simulink model "My_gfm_battery_sil_2_2"  (R2018b)
settings: Solver=ode45  StartTime=0.0  StopTime=30  MaxStep=1e-4  RelTol=1e-3
PreLoadFcn:
  | modelDir = fileparts(get_param(bdroot,'FileName'));
  | 
  | load_system(fullfile(modelDir,'controls_element_lib.slx'));
  | load_system(fullfile(modelDir,'test_sequence_lib.slx'));
InitFcn:
  | close all;
  | clear all;
  | clc;
  | 
  | % frequency nominals
  | F_NOM = 60;
  | W_NOM = 2 * pi * F_NOM;
  | 
  | % base values relative to inverter
  | % --------------------------------
  | VLL_INV_NOM = 480;
  | P_INV_NOM = 1e6;
  | Q_INV_NOM = 0.5e6;
  | S_INV_NOM = sqrt(P_INV_NOM^2 + Q_INV_NOM^2);
  | 
  | I_INV_BASE = S_INV_NOM/(sqrt(3)*VLL_INV_NOM);
  | Z_INV_BASE = VLL_INV_NOM^2/S_INV_NOM;
  | L_INV_BASE = Z_INV_BASE / W_NOM;
  | C_INV_BASE = 1 / (Z_INV_BASE * W_NOM);
  | 
  | % nominal ratings for Plant model
  | % --------------------------------------
  | INVERTER_COUNT = 100;
  | 
  | VLV_NOM = VLL_INV_NOM;
  | VMV_NOM = 35e3;
  | VHV_NOM = 230e3;
  | S_PLANT = INVERTER_COUNT * S_INV_NOM;
  | 
  | N_GSU = VHV_NOM/VMV_NOM;
  | N_MVT = VMV_NOM/VLV_NOM;
  | 
  | I_LV_BASE = S_PLANT/(sqrt(3)*VLV_NOM);
  | I_MV_BASE = S_PLANT/(sqrt(3)*VMV_NOM);
  | I_HV_BASE = S_PLANT/(sqrt(3)*VHV_NOM);
  | 
  | Z_LV_BASE = VLV_NOM^2/S_PLANT;
  | Z_MV_BASE = VMV_NOM^2/S_PLANT;
  | Z_HV_BASE = VHV_NOM^2/S_PLANT;
  | 
  | L_LV_BASE = Z_LV_BASE / W_NOM;
  | L_MV_BASE = Z_MV_BASE / W_NOM;
  | L_HV_BASE = Z_HV_BASE / W_NOM;
  | C_LV_BASE = 1 / (Z_LV_BASE * W_NOM);
  | C_MV_BASE = 1 / (Z_MV_BASE * W_NOM);
  | C_HV_BASE = 1 / (Z_HV_BASE * W_NOM);
  | 
  | % nominal ratings for Grid model
  | % --------------------------------------
  | VGRID_NOM = VHV_NOM;
  | S_GRID = 2*S_PLANT;
  | I_HV_BASE = S_GRID/(sqrt(3)*VGRID_NOM);
  | Z_GRID_BASE = VGRID_NOM^2/S_GRID;
  | L_GRID_BASE = Z_GRID_BASE / W_NOM;
  | C_GRID_BASE = 1 / (Z_GRID_BASE * W_NOM);
undefined symbols (not defined in the file): j
libraries: simulink x74, controls_element_lib x20, test_sequence_lib x12
(part 9 of 9)

== system My_gfm_battery_sil_2_2/My Inverter Controller 1/My_machineModel_A1/rotor model ==
  p_mechanical : Inport
  p_electrical : Inport  Port=2
  Constant : Constant  Value=nominalFrequency
  HPF (wDamperDecoupler) : TransferFcn  Commented=on  Numerator=[0.3 0]  Denominator=[0.3 1]
  HPF (wDamperDecoupler) 1 : Subsystem
  Integrator1 : Integrator  LimitOutput=on  UpperSaturationLimit=5  LowerSaturationLimit=-5
  Sum : Sum  Inputs=++|
  Sum2 : Sum  Inputs=|+-
  Sum3 : Sum  Inputs=|+-
  k_damp : Gain  Gain=kDamper*SRated
  k_inertia : Gain  Gain=(nominalFrequency/2)/(inertialConstant*SRated)
  oscillator_3ph : Subsystem
  osc[3] : Outport  VectorParamsAs1DForOutWhenUnconnected=on
  f_rotor : Outport  Port=2  VectorParamsAs1DForOutWhenUnconnected=on
  wires:
  Constant/1 -> Sum/1
  Sum/1 -> oscillator_3ph/1(f), f_rotor/1
  k_damp/1 -> Sum2/2
  Integrator1/1 -> HPF (wDamperDecoupler) 1/1(in), Sum/2
  p_mechanical/1 -> Sum3/1
  Sum3/1 -> Sum2/1
  p_electrical/1 -> Sum3/2
  HPF (wDamperDecoupler) 1/1(out) -> k_damp/1
  oscillator_3ph/1(osc[3]) -> osc[3]/1
  k_inertia/1 -> Integrator1/1
  Sum2/1 -> k_inertia/1

== system My_gfm_battery_sil_2_2/My Inverter Controller 1/My_machineModel_A1/voltage analyzer ==
  osc[3] : Inport
  v_terminal : Inport  Port=2
  Complex to Magnitude-Angle : ComplexToMagnitudeAngle
  Complex to Real-Imag : ComplexToRealImag
  Conj : Math  Operator=conj  SaturateOnIntegerOverflow=on
  Product1 : Product
  Product2 : Product
  Real-Imag to Complex1 : RealImagToComplex
  Sum of Elements1 : Sum  Inputs=+
  Sum of Elements2 : Sum  Inputs=+
  Terminator : Terminator
  Transfer Fcn : TransferFcn  Denominator=[0.02 1]
  Transfer Fcn1 : TransferFcn  Denominator=[0.02 1]
  over_sqrt(3) : Gain  Gain=1/sqrt(3)
  over_sqrt(3)1 : Gain  Gain=1/sqrt(3)
  sqrt(2) : Gain  Gain=sqrt(2)
  Vd : Outport  VectorParamsAs1DForOutWhenUnconnected=on
  Vq : Outport  Port=2  VectorParamsAs1DForOutWhenUnconnected=on
  Vt_Mag : Outport  Port=3  VectorParamsAs1DForOutWhenUnconnected=on
  wires:
  Transfer Fcn/1 -> Real-Imag to Complex1/2, Vq/1  "Vq"
  osc[3]/1 -> Conj/1
  Transfer Fcn1/1 -> Real-Imag to Complex1/1, Vd/1  "Vd"
  over_sqrt(3)1/1 -> Transfer Fcn1/1
  over_sqrt(3)/1 -> Transfer Fcn/1
  Complex to Real-Imag/1 -> Product2/1
  Complex to Real-Imag/2 -> Product1/1
  Sum of Elements2/1 -> over_sqrt(3)1/1
  v_terminal/1 -> Product2/2, Product1/2
  Product1/1 -> Sum of Elements1/1
  Sum of Elements1/1 -> over_sqrt(3)/1
  sqrt(2)/1 -> Complex to Real-Imag/1
  Conj/1 -> sqrt(2)/1
  Product2/1 -> Sum of Elements2/1
  Complex to Magnitude-Angle/1 -> Vt_Mag/1  "Vt"
  Real-Imag to Complex1/1 -> Complex to Magnitude-Angle/1  "Vd"
  Complex to Magnitude-Angle/2 -> Terminator/1

== system My_gfm_battery_sil_2_2/ac Network with MVT (native math)/OLTC/LPF3 ==
  1 : Inport
  1/10 : Gain  Gain=1/10
  Integrator : Integrator  InitialCondition=1
  Sum4 : Sum  Inputs=|+-
  Out1 : Outport  VectorParamsAs1DForOutWhenUnconnected=on
  wires:
  1/10/1 -> Integrator/1
  Integrator/1 -> Sum4/2, Out1/1
  1/1 -> Sum4/1
  Sum4/1 -> 1/10/1

== system My_gfm_battery_sil_2_2/ac Network with MVT (native math)/OLTC1/LPF3 ==
  1 : Inport
  1/10 : Gain  Gain=1/10
  Integrator : Integrator  InitialCondition=1
  Sum4 : Sum  Inputs=|+-
  Out1 : Outport  VectorParamsAs1DForOutWhenUnconnected=on
  wires:
  1/10/1 -> Integrator/1
  Integrator/1 -> Sum4/2, Out1/1
  1/1 -> Sum4/1
  Sum4/1 -> 1/10/1

== system My_gfm_battery_sil_2_2/My Inverter Controller /My_acMonitor_A/Analyzer_V/complex_LPF ==
  note: This was needed because Simulink complains when using transfer functions directly on arrays or complex numbers.
  In1 : Inport
  Complex to Real-Imag : ComplexToRealImag
  Gain2 : Gain  Gain=1/tau
  Gain3 : Gain  Gain=1/tau
  Integrator : Integrator
  Integrator1 : Integrator
  Real-Imag to Complex : RealImagToComplex
  Sum : Sum  Inputs=|+-
  Sum1 : Sum  Inputs=|+-
  Out1 : Outport  VectorParamsAs1DForOutWhenUnconnected=on
  wires:
  Real-Imag to Complex/1 -> Out1/1
  In1/1 -> Complex to Real-Imag/1
  Complex to Real-Imag/1 -> Sum/1
  Integrator/1 -> Real-Imag to Complex/1, Sum/2
  Sum1/1 -> Gain3/1
  Complex to Real-Imag/2 -> Sum1/1
  Gain2/1 -> Integrator/1
  Sum/1 -> Gain2/1
  Integrator1/1 -> Sum1/2, Real-Imag to Complex/2
  Gain3/1 -> Integrator1/1

== system My_gfm_battery_sil_2_2/My Inverter Controller /My_acMonitor_A/Analyzer_V1/complex_LPF ==
  note: This was needed because Simulink complains when using transfer functions directly on arrays or complex numbers.
  In1 : Inport
  Complex to Real-Imag : ComplexToRealImag
  Gain2 : Gain  Gain=1/tau
  Gain3 : Gain  Gain=1/tau
  Integrator : Integrator
  Integrator1 : Integrator
  Real-Imag to Complex : RealImagToComplex
  Sum : Sum  Inputs=|+-
  Sum1 : Sum  Inputs=|+-
  Out1 : Outport  VectorParamsAs1DForOutWhenUnconnected=on
  wires:
  Real-Imag to Complex/1 -> Out1/1
  In1/1 -> Complex to Real-Imag/1
  Complex to Real-Imag/1 -> Sum/1
  Integrator/1 -> Real-Imag to Complex/1, Sum/2
  Sum1/1 -> Gain3/1
  Complex to Real-Imag/2 -> Sum1/1
  Gain2/1 -> Integrator/1
  Sum/1 -> Gain2/1
  Integrator1/1 -> Sum1/2, Real-Imag to Complex/2
  Gain3/1 -> Integrator1/1

== system My_gfm_battery_sil_2_2/My Inverter Controller /My_acMonitor_A/PLL_3ph/oscillator_3ph ==
  f : Inport
  Cos : Trigonometry  Operator=cos
  Gain : Gain  Gain=2*pi
  Integrator : Integrator
  Real-Imag to Complex : RealImagToComplex
  Sin : Trigonometry
  Sum1 : Sum  Inputs=|++
  phase_shift : Constant  Value=[0 -1/3 -2/3]
  osc[3] : Outport  VectorParamsAs1DForOutWhenUnconnected=on
  wires:
  Sum1/1 -> Gain/1
  phase_shift/1 -> Sum1/2
  Sin/1 -> Real-Imag to Complex/2
  Integrator/1 -> Sum1/1
  Gain/1 -> Sin/1, Cos/1
  Cos/1 -> Real-Imag to Complex/1
  Real-Imag to Complex/1 -> osc[3]/1
  f/1 -> Integrator/1

== system My_gfm_battery_sil_2_2/My Inverter Controller /My_currentLimiting_B/Current_foldback1/LPF  ==
  In : Inport
  1/0.01 : Gain  Gain=1/0.01
  Integrator : Integrator
  Sum3 : Sum  Inputs=|+-
  Out : Outport  VectorParamsAs1DForOutWhenUnconnected=on
  wires:
  Integrator/1 -> Out/1, Sum3/2
  Sum3/1 -> 1/0.01/1
  In/1 -> Sum3/1
  1/0.01/1 -> Integrator/1

== system My_gfm_battery_sil_2_2/My Inverter Controller /My_machineModel_A/AVR/ Saturation ==
  In : Inport
  Complex to Real-Imag : ComplexToRealImag
  Real-Imag to Complex3 : RealImagToComplex
  Saturation3 : Saturate  UpperLimit=0.1*VllRated  LowerLimit=-0.1*VllRated
  Saturation4 : Saturate  UpperLimit=0.1*VllRated  LowerLimit=-0.1*VllRated
  Out : Outport
  wires:
  Complex to Real-Imag/1 -> Saturation3/1
  Saturation4/1 -> Real-Imag to Complex3/2
  Complex to Real-Imag/2 -> Saturation4/1
  Saturation3/1 -> Real-Imag to Complex3/1
  In/1 -> Complex to Real-Imag/1
  Real-Imag to Complex3/1 -> Out/1

== system My_gfm_battery_sil_2_2/My Inverter Controller /My_machineModel_A/AVR/LPF ==
  In : Inport
  1/tauMeas : Gain  Gain=1/tauMeas
  Integrator : Integrator
  Sum3 : Sum  Inputs=|+-
  Out : Outport  VectorParamsAs1DForOutWhenUnconnected=on
  wires:
  Integrator/1 -> Out/1, Sum3/2
  Sum3/1 -> 1/tauMeas/1
  In/1 -> Sum3/1
  1/tauMeas/1 -> Integrator/1

== system My_gfm_battery_sil_2_2/My Inverter Controller /My_machineModel_A/AVR/LPF  ==
  In : Inport
  1/tauMeas : Gain  Gain=1/tauMeas
  Integrator : Integrator
  Sum3 : Sum  Inputs=|+-
  Out : Outport  VectorParamsAs1DForOutWhenUnconnected=on
  wires:
  Integrator/1 -> Out/1, Sum3/2
  Sum3/1 -> 1/tauMeas/1
  In/1 -> Sum3/1
  1/tauMeas/1 -> Integrator/1

== system My_gfm_battery_sil_2_2/My Inverter Controller /My_machineModel_A/AVR/LPF   ==
  In : Inport
  1/tauMeas : Gain  Gain=1/tauMeas
  Integrator : Integrator
  Sum3 : Sum  Inputs=|+-
  Out : Outport  VectorParamsAs1DForOutWhenUnconnected=on
  wires:
  Integrator/1 -> Out/1, Sum3/2
  Sum3/1 -> 1/tauMeas/1
  In/1 -> Sum3/1
  1/tauMeas/1 -> Integrator/1

== system My_gfm_battery_sil_2_2/My Inverter Controller /My_machineModel_A/AVR/assymmetric filter ==
  note: The saturation block is configured to cause a rapid rise, but much slow drop in output.
  in : Inport
  Gain1 : Gain  Gain=1/tauBkSt
  Integrator : Integrator
  Saturation1 : Saturate  UpperLimit=VllRated  LowerLimit=-0.02 * VllRated
  Sum3 : Sum  Inputs=|+-
  out : Outport  VectorParamsAs1DForOutWhenUnconnected=on
  wires:
  Saturation1/1 -> Integrator/1
  Gain1/1 -> Saturation1/1
  in/1 -> Sum3/1
  Sum3/1 -> Gain1/1
  Integrator/1 -> Sum3/2, out/1

== system My_gfm_battery_sil_2_2/My Inverter Controller /My_machineModel_A/AVR/current analyzer ==
  osc[3] : Inport
  iac : Inport  Port=2
  Complex to Real-Imag : ComplexToRealImag
  Conj : Math  Operator=conj  SaturateOnIntegerOverflow=on
  Product1 : Product
  Product2 : Product
  Sum of Elements1 : Sum  Inputs=+
  Sum of Elements2 : Sum  Inputs=+
  Transfer Fcn : TransferFcn  Denominator=[0.02 1]
  Transfer Fcn1 : TransferFcn  Denominator=[0.02 1]
  over_sqrt(3) : Gain  Gain=1/sqrt(3)
  over_sqrt(3)1 : Gain  Gain=1/sqrt(3)
  sqrt(2) : Gain  Gain=sqrt(2)
  Id : Outport  VectorParamsAs1DForOutWhenUnconnected=on
  Iq : Outport  Port=2  VectorParamsAs1DForOutWhenUnconnected=on
  wires:
  Transfer Fcn/1 -> Iq/1
  osc[3]/1 -> Conj/1
  Transfer Fcn1/1 -> Id/1
  over_sqrt(3)1/1 -> Transfer Fcn1/1
  over_sqrt(3)/1 -> Transfer Fcn/1
  Complex to Real-Imag/1 -> Product2/1
  Complex to Real-Imag/2 -> Product1/1
  Sum of Elements2/1 -> over_sqrt(3)1/1
  iac/1 -> Product2/2, Product1/2
  Product1/1 -> Sum of Elements1/1
  Sum of Elements1/1 -> over_sqrt(3)/1
  sqrt(2)/1 -> Complex to Real-Imag/1
  Conj/1 -> sqrt(2)/1
  Product2/1 -> Sum of Elements2/1

== system My_gfm_battery_sil_2_2/My Inverter Controller /My_machineModel_A/Exciter/LPF ==
  In : Inport
  Integrator : Integrator
  Sum3 : Sum  Inputs=|+-
  wExciter : Gain  Gain=wExciter
  Out : Outport  VectorParamsAs1DForOutWhenUnconnected=on
  wires:
  Integrator/1 -> Out/1, Sum3/2
  Sum3/1 -> wExciter/1
  In/1 -> Sum3/1
  wExciter/1 -> Integrator/1

== system My_gfm_battery_sil_2_2/My Inverter Controller /My_machineModel_A/Exciter/modulator ==
  cmd : Inport
  osc : Inport  Port=2
  Complex to Real-Imag : ComplexToRealImag
  Complex to Real-Imag1 : ComplexToRealImag
  Gain : Gain  Gain=sqrt(2)
  Product1 : Product
  Product2 : Product
  Sum1 : Sum  Inputs=|+-
  ref : Outport  VectorParamsAs1DForOutWhenUnconnected=on
  wires:
  osc/1 -> Gain/1
  Complex to Real-Imag/1 -> Product2/2
  Product2/1 -> Sum1/1
  Sum1/1 -> ref/1  "i"
  Gain/1 -> Complex to Real-Imag/1
  Complex to Real-Imag/2 -> Product1/2
  Product1/1 -> Sum1/2
  cmd/1 -> Complex to Real-Imag1/1
  Complex to Real-Imag1/1 -> Product2/1
  Complex to Real-Imag1/2 -> Product1/1

== system My_gfm_battery_sil_2_2/My Inverter Controller /My_machineModel_A/governer/LPF(DamperDecoupler) limited  ==
  In : Inport
  Constant : Constant  Value=1/tau_damp
  Constant1 : Constant  Value=wGoverner
  Integrator : Integrator  LimitOutput=on  UpperSaturationLimit=1.2*SRated  LowerSaturationLimit=-1.2*SRated
  MinMax : MinMax  Inputs=2
  Product : Product
  Sum3 : Sum  Inputs=|+-
  Out : Outport  VectorParamsAs1DForOutWhenUnconnected=on
  wires:
  Integrator/1 -> Out/1, Sum3/2
  Sum3/1 -> Product/2
  In/1 -> Sum3/1
  Product/1 -> Integrator/1
  MinMax/1 -> Product/1
  Constant/1 -> MinMax/1
  Constant1/1 -> MinMax/2

== system My_gfm_battery_sil_2_2/My Inverter Controller /My_machineModel_A/governer/synchronizer ==
  note: Big Range?
  note: prevent it from acting during typical faults
  note: Prevent loss of sync at low voltage events, using asym filter to traget long extended low voltage events
  note: Keeps the machine spining in synchronize while machine is disabled, disabling the machine means
  note: Why?
  Vq : Inport
  Vt : Inport  Port=2
  machine_enabled : Inport  Port=3
  Constant : Constant
  Gain : Gain  Gain=SRated
  Gain2 : Gain  Gain=1/VllRated
  "HPF " : Subsystem
  Product1 : Product
  Saturation : Saturate  UpperLimit=1  LowerLimit=0
  Sum : Sum  Inputs=|++
  Sum2 : Sum  Inputs=|+-
  Switch : Switch  Criteria=u2 > Threshold
  assymmetric filter1 : Subsystem
  gain : Gain  Gain=wSync
  kFastSync : Gain  Gain=kpFastSync
  kSync : Gain  Gain=kpSync
  pSyncLimit : Saturate  UpperLimit=3  LowerLimit=-3
  syncFadeGain : Gain  Gain=kpSyncFade
  syncFadeThreshold : Constant  Value=SyncFadeThres
  to_pu : Gain  Gain=1 / VllRated
  p_sync_pu : Outport  VectorParamsAs1DForOutWhenUnconnected=on
  wires:
  to_pu/1 -> Sum2/2
  Vt/1 -> assymmetric filter1/1(in)
  assymmetric filter1/1(out) -> to_pu/1
  pSyncLimit/1 -> Gain/1
  kSync/1 -> Sum/1
  Sum/1 -> pSyncLimit/1
  Product1/1 -> p_sync_pu/1
  Constant/1 -> Switch/3
  Sum2/1 -> syncFadeGain/1
  machine_enabled/1 -> Switch/2
  syncFadeGain/1 -> Saturation/1
  Saturation/1 -> Switch/1
  syncFadeThreshold/1 -> Sum2/1
  Switch/1 -> Product1/2
  Gain2/1 -> kFastSync/1, kSync/1
  Vq/1 -> Gain2/1
  Gain/1 -> Product1/1  "p_sync"
  kFastSync/1 -> "HPF "/1(in)
  "HPF "/1(out) -> gain/1
  gain/1 -> Sum/2

== system My_gfm_battery_sil_2_2/My Inverter Controller /My_machineModel_A/rotor model/HPF (wDamperDecoupler) 1 ==
  in : Inport
  1/tau_damp : Gain  Gain=1/tau_damp
  Integrator : Integrator
  Sum : Sum  Inputs=|+-
  out : Outport  VectorParamsAs1DForOutWhenUnconnected=on
  wires:
  Sum/1 -> out/1, 1/tau_damp/1
  in/1 -> Sum/1
  Integrator/1 -> Sum/2
  1/tau_damp/1 -> Integrator/1

== system My_gfm_battery_sil_2_2/My Inverter Controller /My_machineModel_A/rotor model/oscillator_3ph ==
  f : Inport
  Cos : Trigonometry  Operator=cos
  Gain : Gain  Gain=2*pi
  Integrator : Integrator
  Real-Imag to Complex : RealImagToComplex
  Sin : Trigonometry
  Sum1 : Sum  Inputs=|++
  phase_shift : Constant  Value=[0 -1/3 -2/3]
  osc[3] : Outport  VectorParamsAs1DForOutWhenUnconnected=on
  wires:
  f/1 -> Integrator/1
  Real-Imag to Complex/1 -> osc[3]/1
  Cos/1 -> Real-Imag to Complex/1
  Gain/1 -> Cos/1, Sin/1
  Integrator/1 -> Sum1/1
  Sin/1 -> Real-Imag to Complex/2
  phase_shift/1 -> Sum1/2
  Sum1/1 -> Gain/1

== system My_gfm_battery_sil_2_2/My Inverter Controller /My_machineModel_A/voltage analyzer/LPF ==
  In : Inport
  1/tauMeas : Gain  Gain=1/tauMeas
  Integrator : Integrator
  Sum3 : Sum  Inputs=|+-
  Out : Outport  VectorParamsAs1DForOutWhenUnconnected=on
  wires:
  Integrator/1 -> Out/1, Sum3/2
  Sum3/1 -> 1/tauMeas/1
  In/1 -> Sum3/1
  1/tauMeas/1 -> Integrator/1

== system My_gfm_battery_sil_2_2/My Inverter Controller /My_machineModel_A/voltage analyzer/LPF  ==
  In : Inport
  1/tauMeas : Gain  Gain=1/tauMeas
  Integrator : Integrator
  Sum3 : Sum  Inputs=|+-
  Out : Outport  VectorParamsAs1DForOutWhenUnconnected=on
  wires:
  Integrator/1 -> Out/1, Sum3/2
  Sum3/1 -> 1/tauMeas/1
  In/1 -> Sum3/1
  1/tauMeas/1 -> Integrator/1

== system My_gfm_battery_sil_2_2/My Inverter Controller /My_machineModel_A1/excitation/LPF ==
  In : Inport
  Integrator : Integrator
  Sum3 : Sum  Inputs=|+-
  wExciter : Gain  Gain=wExciter
  Out : Outport  VectorParamsAs1DForOutWhenUnconnected=on
  wires:
  Integrator/1 -> Out/1, Sum3/2
  Sum3/1 -> wExciter/1
  In/1 -> Sum3/1
  wExciter/1 -> Integrator/1

== system My_gfm_battery_sil_2_2/My Inverter Controller /My_machineModel_A1/excitation/assymmetric filter1 ==
  note: The saturation block is configured to cause a rapid rise, but much slow drop in output.
  in : Inport
  Gain1 : Gain  Gain=2
  Integrator : Integrator
  Saturation1 : Saturate  UpperLimit=VllRated  LowerLimit=-0.02 * VllRated
  Sum3 : Sum  Inputs=|+-
  out : Outport  VectorParamsAs1DForOutWhenUnconnected=on
  wires:
  Saturation1/1 -> Integrator/1
  Gain1/1 -> Saturation1/1
  in/1 -> Sum3/1
  Sum3/1 -> Gain1/1
  Integrator/1 -> Sum3/2, out/1

== system My_gfm_battery_sil_2_2/My Inverter Controller /My_machineModel_A1/excitation/modulator ==
  cmd : Inport
  osc : Inport  Port=2
  Complex to Real-Imag : ComplexToRealImag
  Complex to Real-Imag1 : ComplexToRealImag
  Gain : Gain  Gain=sqrt(2)
  Product1 : Product
  Product2 : Product
  Sum1 : Sum  Inputs=|+-
  ref : Outport  VectorParamsAs1DForOutWhenUnconnected=on
  wires:
  osc/1 -> Gain/1
  Complex to Real-Imag/1 -> Product2/2
  Product2/1 -> Sum1/1
  Sum1/1 -> ref/1  "i"
  Gain/1 -> Complex to Real-Imag/1
  Complex to Real-Imag/2 -> Product1/2
  Product1/1 -> Sum1/2
  cmd/1 -> Complex to Real-Imag1/1
  Complex to Real-Imag1/1 -> Product2/1
  Complex to Real-Imag1/2 -> Product1/1

== system My_gfm_battery_sil_2_2/My Inverter Controller /My_machineModel_A1/governer/LPF(DamperDecoupler) limited  ==
  In : Inport
  1/tau_damp : Gain  Gain=1/0.3
  Integrator : Integrator  LimitOutput=on  UpperSaturationLimit=1.2*SRated  LowerSaturationLimit=-1.2*SRated
  Sum3 : Sum  Inputs=|+-
  Out : Outport  VectorParamsAs1DForOutWhenUnconnected=on
  wires:
  Integrator/1 -> Out/1, Sum3/2
  Sum3/1 -> 1/tau_damp/1
  In/1 -> Sum3/1
  1/tau_damp/1 -> Integrator/1

== system My_gfm_battery_sil_2_2/My Inverter Controller /My_machineModel_A1/governer/synchronizer ==
  note: Why?
  note: Big Range?
  note: prevent it from acting during typical faults
  note: Prevent loss of sync at low voltage events, using asym filter to traget long extended low voltage events
  note: Keeps the machine spining in synchronize while machine is disabled, disabling the machine means
  note: Why?
  Vq : Inport
  Vt : Inport  Port=2
  machine_enabled : Inport  Port=3
  Constant : Constant
  Gain : Gain  Gain=SRated
  Gain2 : Gain  Gain=1/VllRated
  HPF : Subsystem
  Product1 : Product
  Saturation : Saturate  UpperLimit=1  LowerLimit=0
  Sum : Sum  Inputs=|++
  Sum2 : Sum  Inputs=|+-
  Switch : Switch  Criteria=u2 > Threshold
  Transfer Fcn : TransferFcn  Commented=on  Numerator=[(2 * pi * 50) 0]  Denominator=[1, (2*pi*50)]
  assymmetric filter1 : Subsystem
  gain : Gain  Gain=2*pi*50
  kFastSync : Gain
  kSync : Gain  Gain=20
  pSyncLimit : Saturate  UpperLimit=3  LowerLimit=-3
  syncFadeGain : Gain  Gain=4
  syncFadeThreshold : Constant  Value=0.2
  to_pu : Gain  Gain=1 / VllRated
  p_sync_pu : Outport  VectorParamsAs1DForOutWhenUnconnected=on
  wires:
  to_pu/1 -> Sum2/2
  Vt/1 -> assymmetric filter1/1(in)
  assymmetric filter1/1(out) -> to_pu/1
  pSyncLimit/1 -> Gain/1
  kSync/1 -> Sum/1
  Sum/1 -> pSyncLimit/1
  Product1/1 -> p_sync_pu/1
  Constant/1 -> Switch/3
  Sum2/1 -> syncFadeGain/1
  machine_enabled/1 -> Switch/2
  syncFadeGain/1 -> Saturation/1
  Saturation/1 -> Switch/1
  syncFadeThreshold/1 -> Sum2/1
  Switch/1 -> Product1/2
  Gain2/1 -> kFastSync/1, kSync/1
  Vq/1 -> Gain2/1
  Gain/1 -> Product1/1  "p_sync"
  kFastSync/1 -> HPF/1(in)
  HPF/1(out) -> gain/1
  gain/1 -> Sum/2

== system My_gfm_battery_sil_2_2/My Inverter Controller /My_machineModel_A1/governer1/LPF(DamperDecoupler) - limited ==
  In1 : Inport
  Integrator : Integrator  LimitOutput=on  UpperSaturationLimit=1.2*SRated  LowerSaturationLimit=-1.2*SRated
  Sum3 : Sum  Inputs=|+-
  wDamperDecoupler : Gain  Gain=1/0.3
  Out1 : Outport  VectorParamsAs1DForOutWhenUnconnected=on
  wires:
  Integrator/1 -> Out1/1, Sum3/2
  Sum3/1 -> wDamperDecoupler/1
  wDamperDecoupler/1 -> Integrator/1
  In1/1 -> Sum3/1

== system My_gfm_battery_sil_2_2/My Inverter Controller /My_machineModel_A1/governer1/LPF(DamperDecoupler) limited 1 ==
  In : Inport
  1/tau_damp : Gain  Gain=1/0.3
  Integrator : Integrator  LimitOutput=on  UpperSaturationLimit=1.2*SRated  LowerSaturationLimit=-1.2*SRated
  Sum3 : Sum  Inputs=|+-
  Out : Outport  VectorParamsAs1DForOutWhenUnconnected=on
  wires:
  Integrator/1 -> Out/1, Sum3/2
  Sum3/1 -> 1/tau_damp/1
  In/1 -> Sum3/1
  1/tau_damp/1 -> Integrator/1

== system My_gfm_battery_sil_2_2/My Inverter Controller /My_machineModel_A1/governer1/synchronizer ==
  note: Why?
  note: Big Range?
  note: prevent it from acting during typical faults
  note: Prevent loss of sync at low voltage events, using asym filter to traget long extended low voltage events
  note: Keeps the machine spining in synchronize while machine is disabled, disabling the machine means
  note: Why?
  note: Should be sqrt(Vd^2 + Vq^2) ?
  Vq : Inport
  Vd : Inport  Port=2
  machine_enabled : Inport  Port=3
  Constant : Constant
  Gain : Gain  Gain=SRated
  Gain2 : Gain  Gain=1/VllRated
  HPF : Subsystem
  Product1 : Product
  Saturation : Saturate  UpperLimit=1  LowerLimit=0
  Sum : Sum  Inputs=|++
  Sum2 : Sum  Inputs=|+-
  Switch : Switch  Criteria=u2 > Threshold
  Transfer Fcn : TransferFcn  Commented=on  Numerator=[(2 * pi * 50) 0]  Denominator=[1, (2*pi*50)]
  assymmetric filter1 : Subsystem
  gain : Gain  Gain=2*pi*50
  kFastSync : Gain
  kSync : Gain  Gain=20
  pSyncLimit : Saturate  UpperLimit=3  LowerLimit=-3
  syncFadeGain : Gain  Gain=4
  syncFadeThreshold : Constant  Value=0.2
  to_pu : Gain  Gain=1 / VllRated
  p_sync_pu : Outport  VectorParamsAs1DForOutWhenUnconnected=on
  wires:
  to_pu/1 -> Sum2/2
  Vd/1 -> assymmetric filter1/1(in)
  assymmetric filter1/1(out) -> to_pu/1
  pSyncLimit/1 -> Gain/1
  kSync/1 -> Sum/1
  Sum/1 -> pSyncLimit/1
  Product1/1 -> p_sync_pu/1
  Constant/1 -> Switch/3
  Sum2/1 -> syncFadeGain/1
  machine_enabled/1 -> Switch/2
  syncFadeGain/1 -> Saturation/1
  Saturation/1 -> Switch/1
  syncFadeThreshold/1 -> Sum2/1
  Switch/1 -> Product1/2
  Gain2/1 -> kFastSync/1, kSync/1
  Vq/1 -> Gain2/1
  Gain/1 -> Product1/1  "p_sync"
  kFastSync/1 -> HPF/1(in)
  HPF/1(out) -> gain/1
  gain/1 -> Sum/2

== system My_gfm_battery_sil_2_2/My Inverter Controller /My_machineModel_A1/rotor model/HPF (wDamperDecoupler) 1 ==
  in : Inport
  1/tau_damp : Gain  Gain=1/0.3
  Integrator : Integrator
  Sum : Sum  Inputs=|+-
  out : Outport  VectorParamsAs1DForOutWhenUnconnected=on
  wires:
  Sum/1 -> out/1, 1/tau_damp/1
  in/1 -> Sum/1
  Integrator/1 -> Sum/2
  1/tau_damp/1 -> Integrator/1

== system My_gfm_battery_sil_2_2/My Inverter Controller /My_machineModel_A1/rotor model/oscillator_3ph ==
  f : Inport
  Cos : Trigonometry  Operator=cos
  Gain : Gain  Gain=2*pi
  Integrator : Integrator
  Real-Imag to Complex : RealImagToComplex
  Sin : Trigonometry
  Sum1 : Sum  Inputs=|++
  phase_shift : Constant  Value=[0 -1/3 -2/3]
  osc[3] : Outport  VectorParamsAs1DForOutWhenUnconnected=on
  wires:
  f/1 -> Integrator/1
  Real-Imag to Complex/1 -> osc[3]/1
  Cos/1 -> Real-Imag to Complex/1
  Gain/1 -> Cos/1, Sin/1
  Integrator/1 -> Sum1/1
  Sin/1 -> Real-Imag to Complex/2
  phase_shift/1 -> Sum1/2
  Sum1/1 -> Gain/1

== system My_gfm_battery_sil_2_2/My Inverter Controller 1/My_acMonitor_A/Analyzer_V/complex_LPF ==
  note: This was needed because Simulink complains when using transfer functions directly on arrays or complex numbers.
  In1 : Inport
  Complex to Real-Imag : ComplexToRealImag
  Gain2 : Gain  Gain=1/tau
  Gain3 : Gain  Gain=1/tau
  Integrator : Integrator
  Integrator1 : Integrator
  Real-Imag to Complex : RealImagToComplex
  Sum : Sum  Inputs=|+-
  Sum1 : Sum  Inputs=|+-
  Out1 : Outport  VectorParamsAs1DForOutWhenUnconnected=on
  wires:
  Real-Imag to Complex/1 -> Out1/1
  In1/1 -> Complex to Real-Imag/1
  Complex to Real-Imag/1 -> Sum/1
  Integrator/1 -> Real-Imag to Complex/1, Sum/2
  Sum1/1 -> Gain3/1
  Complex to Real-Imag/2 -> Sum1/1
  Gain2/1 -> Integrator/1
  Sum/1 -> Gain2/1
  Integrator1/1 -> Sum1/2, Real-Imag to Complex/2
  Gain3/1 -> Integrator1/1

== system My_gfm_battery_sil_2_2/My Inverter Controller 1/My_acMonitor_A/Analyzer_V1/complex_LPF ==
  note: This was needed because Simulink complains when using transfer functions directly on arrays or complex numbers.
  In1 : Inport
  Complex to Real-Imag : ComplexToRealImag
  Gain2 : Gain  Gain=1/tau
  Gain3 : Gain  Gain=1/tau
  Integrator : Integrator
  Integrator1 : Integrator
  Real-Imag to Complex : RealImagToComplex
  Sum : Sum  Inputs=|+-
  Sum1 : Sum  Inputs=|+-
  Out1 : Outport  VectorParamsAs1DForOutWhenUnconnected=on
  wires:
  Real-Imag to Complex/1 -> Out1/1
  In1/1 -> Complex to Real-Imag/1
  Complex to Real-Imag/1 -> Sum/1
  Integrator/1 -> Real-Imag to Complex/1, Sum/2
  Sum1/1 -> Gain3/1
  Complex to Real-Imag/2 -> Sum1/1
  Gain2/1 -> Integrator/1
  Sum/1 -> Gain2/1
  Integrator1/1 -> Sum1/2, Real-Imag to Complex/2
  Gain3/1 -> Integrator1/1

== system My_gfm_battery_sil_2_2/My Inverter Controller 1/My_acMonitor_A/PLL_3ph/oscillator_3ph ==
  f : Inport
  Cos : Trigonometry  Operator=cos
  Gain : Gain  Gain=2*pi
  Integrator : Integrator
  Real-Imag to Complex : RealImagToComplex
  Sin : Trigonometry
  Sum1 : Sum  Inputs=|++
  phase_shift : Constant  Value=[0 -1/3 -2/3]
  osc[3] : Outport  VectorParamsAs1DForOutWhenUnconnected=on
  wires:
  Sum1/1 -> Gain/1
  phase_shift/1 -> Sum1/2
  Sin/1 -> Real-Imag to Complex/2
  Integrator/1 -> Sum1/1
  Gain/1 -> Sin/1, Cos/1
  Cos/1 -> Real-Imag to Complex/1
  Real-Imag to Complex/1 -> osc[3]/1
  f/1 -> Integrator/1

== system My_gfm_battery_sil_2_2/My Inverter Controller 1/My_currentLimiting_B/Current_foldback1/LPF  ==
  In : Inport
  1/0.01 : Gain  Gain=1/0.01
  Integrator : Integrator
  Sum3 : Sum  Inputs=|+-
  Out : Outport  VectorParamsAs1DForOutWhenUnconnected=on
  wires:
  Integrator/1 -> Out/1, Sum3/2
  Sum3/1 -> 1/0.01/1
  In/1 -> Sum3/1
  1/0.01/1 -> Integrator/1

== system My_gfm_battery_sil_2_2/My Inverter Controller 1/My_machineModel_A/AVR/ Saturation ==
  In : Inport
  Complex to Real-Imag : ComplexToRealImag
  Real-Imag to Complex3 : RealImagToComplex
  Saturation3 : Saturate  UpperLimit=0.1*VllRated  LowerLimit=-0.1*VllRated
  Saturation4 : Saturate  UpperLimit=0.1*VllRated  LowerLimit=-0.1*VllRated
  Out : Outport
  wires:
  Complex to Real-Imag/1 -> Saturation3/1
  Saturation4/1 -> Real-Imag to Complex3/2
  Complex to Real-Imag/2 -> Saturation4/1
  Saturation3/1 -> Real-Imag to Complex3/1
  In/1 -> Complex to Real-Imag/1
  Real-Imag to Complex3/1 -> Out/1

== system My_gfm_battery_sil_2_2/My Inverter Controller 1/My_machineModel_A/AVR/LPF ==
  In : Inport
  1/tauMeas : Gain  Gain=1/tauMeas
  Integrator : Integrator
  Sum3 : Sum  Inputs=|+-
  Out : Outport  VectorParamsAs1DForOutWhenUnconnected=on
  wires:
  Integrator/1 -> Out/1, Sum3/2
  Sum3/1 -> 1/tauMeas/1
  In/1 -> Sum3/1
  1/tauMeas/1 -> Integrator/1

== system My_gfm_battery_sil_2_2/My Inverter Controller 1/My_machineModel_A/AVR/LPF  ==
  In : Inport
  1/tauMeas : Gain  Gain=1/tauMeas
  Integrator : Integrator
  Sum3 : Sum  Inputs=|+-
  Out : Outport  VectorParamsAs1DForOutWhenUnconnected=on
  wires:
  Integrator/1 -> Out/1, Sum3/2
  Sum3/1 -> 1/tauMeas/1
  In/1 -> Sum3/1
  1/tauMeas/1 -> Integrator/1

== system My_gfm_battery_sil_2_2/My Inverter Controller 1/My_machineModel_A/AVR/LPF   ==
  In : Inport
  1/tauMeas : Gain  Gain=1/tauMeas
  Integrator : Integrator
  Sum3 : Sum  Inputs=|+-
  Out : Outport  VectorParamsAs1DForOutWhenUnconnected=on
  wires:
  Integrator/1 -> Out/1, Sum3/2
  Sum3/1 -> 1/tauMeas/1
  In/1 -> Sum3/1
  1/tauMeas/1 -> Integrator/1

== system My_gfm_battery_sil_2_2/My Inverter Controller 1/My_machineModel_A/AVR/assymmetric filter ==
  note: The saturation block is configured to cause a rapid rise, but much slow drop in output.
  in : Inport
  Gain1 : Gain  Gain=1/tauBkSt
  Integrator : Integrator
  Saturation1 : Saturate  UpperLimit=VllRated  LowerLimit=-0.02 * VllRated
  Sum3 : Sum  Inputs=|+-
  out : Outport  VectorParamsAs1DForOutWhenUnconnected=on
  wires:
  Saturation1/1 -> Integrator/1
  Gain1/1 -> Saturation1/1
  in/1 -> Sum3/1
  Sum3/1 -> Gain1/1
  Integrator/1 -> Sum3/2, out/1

== system My_gfm_battery_sil_2_2/My Inverter Controller 1/My_machineModel_A/AVR/current analyzer ==
  osc[3] : Inport
  iac : Inport  Port=2
  Complex to Real-Imag : ComplexToRealImag
  Conj : Math  Operator=conj  SaturateOnIntegerOverflow=on
  Product1 : Product
  Product2 : Product
  Sum of Elements1 : Sum  Inputs=+
  Sum of Elements2 : Sum  Inputs=+
  Transfer Fcn : TransferFcn  Denominator=[0.02 1]
  Transfer Fcn1 : TransferFcn  Denominator=[0.02 1]
  over_sqrt(3) : Gain  Gain=1/sqrt(3)
  over_sqrt(3)1 : Gain  Gain=1/sqrt(3)
  sqrt(2) : Gain  Gain=sqrt(2)
  Id : Outport  VectorParamsAs1DForOutWhenUnconnected=on
  Iq : Outport  Port=2  VectorParamsAs1DForOutWhenUnconnected=on
  wires:
  Transfer Fcn/1 -> Iq/1
  osc[3]/1 -> Conj/1
  Transfer Fcn1/1 -> Id/1
  over_sqrt(3)1/1 -> Transfer Fcn1/1
  over_sqrt(3)/1 -> Transfer Fcn/1
  Complex to Real-Imag/1 -> Product2/1
  Complex to Real-Imag/2 -> Product1/1
  Sum of Elements2/1 -> over_sqrt(3)1/1
  iac/1 -> Product2/2, Product1/2
  Product1/1 -> Sum of Elements1/1
  Sum of Elements1/1 -> over_sqrt(3)/1
  sqrt(2)/1 -> Complex to Real-Imag/1
  Conj/1 -> sqrt(2)/1
  Product2/1 -> Sum of Elements2/1

== system My_gfm_battery_sil_2_2/My Inverter Controller 1/My_machineModel_A/Exciter/LPF ==
  In : Inport
  Integrator : Integrator
  Sum3 : Sum  Inputs=|+-
  wExciter : Gain  Gain=wExciter
  Out : Outport  VectorParamsAs1DForOutWhenUnconnected=on
  wires:
  Integrator/1 -> Out/1, Sum3/2
  Sum3/1 -> wExciter/1
  In/1 -> Sum3/1
  wExciter/1 -> Integrator/1

== system My_gfm_battery_sil_2_2/My Inverter Controller 1/My_machineModel_A/Exciter/modulator ==
  cmd : Inport
  osc : Inport  Port=2
  Complex to Real-Imag : ComplexToRealImag
  Complex to Real-Imag1 : ComplexToRealImag
  Gain : Gain  Gain=sqrt(2)
  Product1 : Product
  Product2 : Product
  Sum1 : Sum  Inputs=|+-
  ref : Outport  VectorParamsAs1DForOutWhenUnconnected=on
  wires:
  osc/1 -> Gain/1
  Complex to Real-Imag/1 -> Product2/2
  Product2/1 -> Sum1/1
  Sum1/1 -> ref/1  "i"
  Gain/1 -> Complex to Real-Imag/1
  Complex to Real-Imag/2 -> Product1/2
  Product1/1 -> Sum1/2
  cmd/1 -> Complex to Real-Imag1/1
  Complex to Real-Imag1/1 -> Product2/1
  Complex to Real-Imag1/2 -> Product1/1

== system My_gfm_battery_sil_2_2/My Inverter Controller 1/My_machineModel_A/governer/LPF(DamperDecoupler) limited  ==
  In : Inport
  Constant : Constant  Value=1/tau_damp
  Constant1 : Constant  Value=wGoverner
  Integrator : Integrator  LimitOutput=on  UpperSaturationLimit=1.2*SRated  LowerSaturationLimit=-1.2*SRated
  MinMax : MinMax  Inputs=2
  Product : Product
  Sum3 : Sum  Inputs=|+-
  Out : Outport  VectorParamsAs1DForOutWhenUnconnected=on
  wires:
  Integrator/1 -> Out/1, Sum3/2
  Sum3/1 -> Product/2
  In/1 -> Sum3/1
  Product/1 -> Integrator/1
  MinMax/1 -> Product/1
  Constant/1 -> MinMax/1
  Constant1/1 -> MinMax/2

== system My_gfm_battery_sil_2_2/My Inverter Controller 1/My_machineModel_A/governer/synchronizer ==
  note: Big Range?
  note: prevent it from acting during typical faults
  note: Prevent loss of sync at low voltage events, using asym filter to traget long extended low voltage events
  note: Keeps the machine spining in synchronize while machine is disabled, disabling the machine means
  note: Why?
  Vq : Inport
  Vt : Inport  Port=2
  machine_enabled : Inport  Port=3
  Constant : Constant
  Gain : Gain  Gain=SRated
  Gain2 : Gain  Gain=1/VllRated
  "HPF " : Subsystem
  Product1 : Product
  Saturation : Saturate  UpperLimit=1  LowerLimit=0
  Sum : Sum  Inputs=|++
  Sum2 : Sum  Inputs=|+-
  Switch : Switch  Criteria=u2 > Threshold
  assymmetric filter1 : Subsystem
  gain : Gain  Gain=wSync
  kFastSync : Gain  Gain=kpFastSync
  kSync : Gain  Gain=kpSync
  pSyncLimit : Saturate  UpperLimit=3  LowerLimit=-3
  syncFadeGain : Gain  Gain=kpSyncFade
  syncFadeThreshold : Constant  Value=SyncFadeThres
  to_pu : Gain  Gain=1 / VllRated
  p_sync_pu : Outport  VectorParamsAs1DForOutWhenUnconnected=on
  wires:
  to_pu/1 -> Sum2/2
  Vt/1 -> assymmetric filter1/1(in)
  assymmetric filter1/1(out) -> to_pu/1
  pSyncLimit/1 -> Gain/1
  kSync/1 -> Sum/1
  Sum/1 -> pSyncLimit/1
  Product1/1 -> p_sync_pu/1
  Constant/1 -> Switch/3
  Sum2/1 -> syncFadeGain/1
  machine_enabled/1 -> Switch/2
  syncFadeGain/1 -> Saturation/1
  Saturation/1 -> Switch/1
  syncFadeThreshold/1 -> Sum2/1
  Switch/1 -> Product1/2
  Gain2/1 -> kFastSync/1, kSync/1
  Vq/1 -> Gain2/1
  Gain/1 -> Product1/1  "p_sync"
  kFastSync/1 -> "HPF "/1(in)
  "HPF "/1(out) -> gain/1
  gain/1 -> Sum/2

== system My_gfm_battery_sil_2_2/My Inverter Controller 1/My_machineModel_A/rotor model/HPF (wDamperDecoupler) 1 ==
  in : Inport
  1/tau_damp : Gain  Gain=1/tau_damp
  Integrator : Integrator
  Sum : Sum  Inputs=|+-
  out : Outport  VectorParamsAs1DForOutWhenUnconnected=on
  wires:
  Sum/1 -> out/1, 1/tau_damp/1
  in/1 -> Sum/1
  Integrator/1 -> Sum/2
  1/tau_damp/1 -> Integrator/1

== system My_gfm_battery_sil_2_2/My Inverter Controller 1/My_machineModel_A/rotor model/oscillator_3ph ==
  f : Inport
  Cos : Trigonometry  Operator=cos
  Gain : Gain  Gain=2*pi
  Integrator : Integrator
  Real-Imag to Complex : RealImagToComplex
  Sin : Trigonometry
  Sum1 : Sum  Inputs=|++
  phase_shift : Constant  Value=[0 -1/3 -2/3]
  osc[3] : Outport  VectorParamsAs1DForOutWhenUnconnected=on
  wires:
  f/1 -> Integrator/1
  Real-Imag to Complex/1 -> osc[3]/1
  Cos/1 -> Real-Imag to Complex/1
  Gain/1 -> Cos/1, Sin/1
  Integrator/1 -> Sum1/1
  Sin/1 -> Real-Imag to Complex/2
  phase_shift/1 -> Sum1/2
  Sum1/1 -> Gain/1

== system My_gfm_battery_sil_2_2/My Inverter Controller 1/My_machineModel_A/voltage analyzer/LPF ==
  In : Inport
  1/tauMeas : Gain  Gain=1/tauMeas
  Integrator : Integrator
  Sum3 : Sum  Inputs=|+-
  Out : Outport  VectorParamsAs1DForOutWhenUnconnected=on
  wires:
  Integrator/1 -> Out/1, Sum3/2
  Sum3/1 -> 1/tauMeas/1
  In/1 -> Sum3/1
  1/tauMeas/1 -> Integrator/1

== system My_gfm_battery_sil_2_2/My Inverter Controller 1/My_machineModel_A/voltage analyzer/LPF  ==
  In : Inport
  1/tauMeas : Gain  Gain=1/tauMeas
  Integrator : Integrator
  Sum3 : Sum  Inputs=|+-
  Out : Outport  VectorParamsAs1DForOutWhenUnconnected=on
  wires:
  Integrator/1 -> Out/1, Sum3/2
  Sum3/1 -> 1/tauMeas/1
  In/1 -> Sum3/1
  1/tauMeas/1 -> Integrator/1

== system My_gfm_battery_sil_2_2/My Inverter Controller 1/My_machineModel_A1/excitation/LPF ==
  In : Inport
  Integrator : Integrator
  Sum3 : Sum  Inputs=|+-
  wExciter : Gain  Gain=wExciter
  Out : Outport  VectorParamsAs1DForOutWhenUnconnected=on
  wires:
  Integrator/1 -> Out/1, Sum3/2
  Sum3/1 -> wExciter/1
  In/1 -> Sum3/1
  wExciter/1 -> Integrator/1

== system My_gfm_battery_sil_2_2/My Inverter Controller 1/My_machineModel_A1/excitation/assymmetric filter1 ==
  note: The saturation block is configured to cause a rapid rise, but much slow drop in output.
  in : Inport
  Gain1 : Gain  Gain=2
  Integrator : Integrator
  Saturation1 : Saturate  UpperLimit=VllRated  LowerLimit=-0.02 * VllRated
  Sum3 : Sum  Inputs=|+-
  out : Outport  VectorParamsAs1DForOutWhenUnconnected=on
  wires:
  Saturation1/1 -> Integrator/1
  Gain1/1 -> Saturation1/1
  in/1 -> Sum3/1
  Sum3/1 -> Gain1/1
  Integrator/1 -> Sum3/2, out/1

== system My_gfm_battery_sil_2_2/My Inverter Controller 1/My_machineModel_A1/excitation/modulator ==
  cmd : Inport
  osc : Inport  Port=2
  Complex to Real-Imag : ComplexToRealImag
  Complex to Real-Imag1 : ComplexToRealImag
  Gain : Gain  Gain=sqrt(2)
  Product1 : Product
  Product2 : Product
  Sum1 : Sum  Inputs=|+-
  ref : Outport  VectorParamsAs1DForOutWhenUnconnected=on
  wires:
  osc/1 -> Gain/1
  Complex to Real-Imag/1 -> Product2/2
  Product2/1 -> Sum1/1
  Sum1/1 -> ref/1  "i"
  Gain/1 -> Complex to Real-Imag/1
  Complex to Real-Imag/2 -> Product1/2
  Product1/1 -> Sum1/2
  cmd/1 -> Complex to Real-Imag1/1
  Complex to Real-Imag1/1 -> Product2/1
  Complex to Real-Imag1/2 -> Product1/1

== system My_gfm_battery_sil_2_2/My Inverter Controller 1/My_machineModel_A1/governer/LPF(DamperDecoupler) limited  ==
  In : Inport
  1/tau_damp : Gain  Gain=1/0.3
  Integrator : Integrator  LimitOutput=on  UpperSaturationLimit=1.2*SRated  LowerSaturationLimit=-1.2*SRated
  Sum3 : Sum  Inputs=|+-
  Out : Outport  VectorParamsAs1DForOutWhenUnconnected=on
  wires:
  Integrator/1 -> Out/1, Sum3/2
  Sum3/1 -> 1/tau_damp/1
  In/1 -> Sum3/1
  1/tau_damp/1 -> Integrator/1

== system My_gfm_battery_sil_2_2/My Inverter Controller 1/My_machineModel_A1/governer/synchronizer ==
  note: Why?
  note: Big Range?
  note: prevent it from acting during typical faults
  note: Prevent loss of sync at low voltage events, using asym filter to traget long extended low voltage events
  note: Keeps the machine spining in synchronize while machine is disabled, disabling the machine means
  note: Why?
  Vq : Inport
  Vt : Inport  Port=2
  machine_enabled : Inport  Port=3
  Constant : Constant
  Gain : Gain  Gain=SRated
  Gain2 : Gain  Gain=1/VllRated
  HPF : Subsystem
  Product1 : Product
  Saturation : Saturate  UpperLimit=1  LowerLimit=0
  Sum : Sum  Inputs=|++
  Sum2 : Sum  Inputs=|+-
  Switch : Switch  Criteria=u2 > Threshold
  Transfer Fcn : TransferFcn  Commented=on  Numerator=[(2 * pi * 50) 0]  Denominator=[1, (2*pi*50)]
  assymmetric filter1 : Subsystem
  gain : Gain  Gain=2*pi*50
  kFastSync : Gain
  kSync : Gain  Gain=20
  pSyncLimit : Saturate  UpperLimit=3  LowerLimit=-3
  syncFadeGain : Gain  Gain=4
  syncFadeThreshold : Constant  Value=0.2
  to_pu : Gain  Gain=1 / VllRated
  p_sync_pu : Outport  VectorParamsAs1DForOutWhenUnconnected=on
  wires:
  to_pu/1 -> Sum2/2
  Vt/1 -> assymmetric filter1/1(in)
  assymmetric filter1/1(out) -> to_pu/1
  pSyncLimit/1 -> Gain/1
  kSync/1 -> Sum/1
  Sum/1 -> pSyncLimit/1
  Product1/1 -> p_sync_pu/1
  Constant/1 -> Switch/3
  Sum2/1 -> syncFadeGain/1
  machine_enabled/1 -> Switch/2
  syncFadeGain/1 -> Saturation/1
  Saturation/1 -> Switch/1
  syncFadeThreshold/1 -> Sum2/1
  Switch/1 -> Product1/2
  Gain2/1 -> kFastSync/1, kSync/1
  Vq/1 -> Gain2/1
  Gain/1 -> Product1/1  "p_sync"
  kFastSync/1 -> HPF/1(in)
  HPF/1(out) -> gain/1
  gain/1 -> Sum/2

== system My_gfm_battery_sil_2_2/My Inverter Controller 1/My_machineModel_A1/governer1/LPF(DamperDecoupler) - limited ==
  In1 : Inport
  Integrator : Integrator  LimitOutput=on  UpperSaturationLimit=1.2*SRated  LowerSaturationLimit=-1.2*SRated
  Sum3 : Sum  Inputs=|+-
  wDamperDecoupler : Gain  Gain=1/0.3
  Out1 : Outport  VectorParamsAs1DForOutWhenUnconnected=on
  wires:
  Integrator/1 -> Out1/1, Sum3/2
  Sum3/1 -> wDamperDecoupler/1
  wDamperDecoupler/1 -> Integrator/1
  In1/1 -> Sum3/1

== system My_gfm_battery_sil_2_2/My Inverter Controller 1/My_machineModel_A1/governer1/LPF(DamperDecoupler) limited 1 ==
  In : Inport
  1/tau_damp : Gain  Gain=1/0.3
  Integrator : Integrator  LimitOutput=on  UpperSaturationLimit=1.2*SRated  LowerSaturationLimit=-1.2*SRated
  Sum3 : Sum  Inputs=|+-
  Out : Outport  VectorParamsAs1DForOutWhenUnconnected=on
  wires:
  Integrator/1 -> Out/1, Sum3/2
  Sum3/1 -> 1/tau_damp/1
  In/1 -> Sum3/1
  1/tau_damp/1 -> Integrator/1

== system My_gfm_battery_sil_2_2/My Inverter Controller 1/My_machineModel_A1/governer1/synchronizer ==
  note: Why?
  note: Big Range?
  note: prevent it from acting during typical faults
  note: Prevent loss of sync at low voltage events, using asym filter to traget long extended low voltage events
  note: Keeps the machine spining in synchronize while machine is disabled, disabling the machine means
  note: Why?
  note: Should be sqrt(Vd^2 + Vq^2) ?
  Vq : Inport
  Vd : Inport  Port=2
  machine_enabled : Inport  Port=3
  Constant : Constant
  Gain : Gain  Gain=SRated
  Gain2 : Gain  Gain=1/VllRated
  HPF : Subsystem
  Product1 : Product
  Saturation : Saturate  UpperLimit=1  LowerLimit=0
  Sum : Sum  Inputs=|++
  Sum2 : Sum  Inputs=|+-
  Switch : Switch  Criteria=u2 > Threshold
  Transfer Fcn : TransferFcn  Commented=on  Numerator=[(2 * pi * 50) 0]  Denominator=[1, (2*pi*50)]
  assymmetric filter1 : Subsystem
  gain : Gain  Gain=2*pi*50
  kFastSync : Gain
  kSync : Gain  Gain=20
  pSyncLimit : Saturate  UpperLimit=3  LowerLimit=-3
  syncFadeGain : Gain  Gain=4
  syncFadeThreshold : Constant  Value=0.2
  to_pu : Gain  Gain=1 / VllRated
  p_sync_pu : Outport  VectorParamsAs1DForOutWhenUnconnected=on
  wires:
  to_pu/1 -> Sum2/2
  Vd/1 -> assymmetric filter1/1(in)
  assymmetric filter1/1(out) -> to_pu/1
  pSyncLimit/1 -> Gain/1
  kSync/1 -> Sum/1
  Sum/1 -> pSyncLimit/1
  Product1/1 -> p_sync_pu/1
  Constant/1 -> Switch/3
  Sum2/1 -> syncFadeGain/1
  machine_enabled/1 -> Switch/2
  syncFadeGain/1 -> Saturation/1
  Saturation/1 -> Switch/1
  syncFadeThreshold/1 -> Sum2/1
  Switch/1 -> Product1/2
  Gain2/1 -> kFastSync/1, kSync/1
  Vq/1 -> Gain2/1
  Gain/1 -> Product1/1  "p_sync"
  kFastSync/1 -> HPF/1(in)
  HPF/1(out) -> gain/1
  gain/1 -> Sum/2

== system My_gfm_battery_sil_2_2/My Inverter Controller 1/My_machineModel_A1/rotor model/HPF (wDamperDecoupler) 1 ==
  in : Inport
  1/tau_damp : Gain  Gain=1/0.3
  Integrator : Integrator
  Sum : Sum  Inputs=|+-
  out : Outport  VectorParamsAs1DForOutWhenUnconnected=on
  wires:
  Sum/1 -> out/1, 1/tau_damp/1
  in/1 -> Sum/1
  Integrator/1 -> Sum/2
  1/tau_damp/1 -> Integrator/1

== system My_gfm_battery_sil_2_2/My Inverter Controller 1/My_machineModel_A1/rotor model/oscillator_3ph ==
  f : Inport
  Cos : Trigonometry  Operator=cos
  Gain : Gain  Gain=2*pi
  Integrator : Integrator
  Real-Imag to Complex : RealImagToComplex
  Sin : Trigonometry
  Sum1 : Sum  Inputs=|++
  phase_shift : Constant  Value=[0 -1/3 -2/3]
  osc[3] : Outport  VectorParamsAs1DForOutWhenUnconnected=on
  wires:
  f/1 -> Integrator/1
  Real-Imag to Complex/1 -> osc[3]/1
  Cos/1 -> Real-Imag to Complex/1
  Gain/1 -> Cos/1, Sin/1
  Integrator/1 -> Sum1/1
  Sin/1 -> Real-Imag to Complex/2
  phase_shift/1 -> Sum1/2
  Sum1/1 -> Gain/1

== system My_gfm_battery_sil_2_2/My Inverter Controller /My_machineModel_A/governer/synchronizer/HPF  ==
  in : Inport
  Integrator : Integrator
  Sum : Sum  Inputs=|+-
  wSync : Gain  Gain=wSync
  out : Outport  VectorParamsAs1DForOutWhenUnconnected=on
  wires:
  Sum/1 -> out/1, wSync/1
  in/1 -> Sum/1
  Integrator/1 -> Sum/2
  wSync/1 -> Integrator/1

== system My_gfm_battery_sil_2_2/My Inverter Controller /My_machineModel_A/governer/synchronizer/assymmetric filter1 ==
  note: The saturation block is configured to cause a rapid rise, but much slow drop in output.
  in : Inport
  Gain1 : Gain  Gain=1/tauBkSt
  Integrator : Integrator
  Saturation1 : Saturate  UpperLimit=VllRated  LowerLimit=-0.02 * VllRated
  Sum3 : Sum  Inputs=|+-
  out : Outport  VectorParamsAs1DForOutWhenUnconnected=on
  wires:
  Integrator/1 -> out/1, Sum3/2
  Sum3/1 -> Gain1/1
  in/1 -> Sum3/1
  Gain1/1 -> Saturation1/1
  Saturation1/1 -> Integrator/1

== system My_gfm_battery_sil_2_2/My Inverter Controller /My_machineModel_A1/governer/synchronizer/HPF ==
  in : Inport
  1/tau : Gain  Gain=2*pi*50
  Integrator : Integrator
  Sum : Sum  Inputs=|+-
  out : Outport  VectorParamsAs1DForOutWhenUnconnected=on
  wires:
  Sum/1 -> out/1, 1/tau/1
  in/1 -> Sum/1
  Integrator/1 -> Sum/2
  1/tau/1 -> Integrator/1

== system My_gfm_battery_sil_2_2/My Inverter Controller /My_machineModel_A1/governer/synchronizer/assymmetric filter1 ==
  note: The saturation block is configured to cause a rapid rise, but much slow drop in output.
  in : Inport
  Gain1 : Gain  Gain=2
  Integrator : Integrator
  Saturation1 : Saturate  UpperLimit=VllRated  LowerLimit=-0.02 * VllRated
  Sum3 : Sum  Inputs=|+-
  out : Outport  VectorParamsAs1DForOutWhenUnconnected=on
  wires:
  Integrator/1 -> out/1, Sum3/2
  Sum3/1 -> Gain1/1
  in/1 -> Sum3/1
  Gain1/1 -> Saturation1/1
  Saturation1/1 -> Integrator/1

== system My_gfm_battery_sil_2_2/My Inverter Controller /My_machineModel_A1/governer1/synchronizer/HPF ==
  in : Inport
  1/tau : Gain  Gain=2*pi*50
  Integrator : Integrator
  Sum : Sum  Inputs=|+-
  out : Outport  VectorParamsAs1DForOutWhenUnconnected=on
  wires:
  Sum/1 -> out/1, 1/tau/1
  in/1 -> Sum/1
  Integrator/1 -> Sum/2
  1/tau/1 -> Integrator/1

== system My_gfm_battery_sil_2_2/My Inverter Controller /My_machineModel_A1/governer1/synchronizer/assymmetric filter1 ==
  note: The saturation block is configured to cause a rapid rise, but much slow drop in output.
  in : Inport
  Gain1 : Gain  Gain=2
  Integrator : Integrator
  Saturation1 : Saturate  UpperLimit=VllRated  LowerLimit=-0.02 * VllRated
  Sum3 : Sum  Inputs=|+-
  out : Outport  VectorParamsAs1DForOutWhenUnconnected=on
  wires:
  Integrator/1 -> out/1, Sum3/2
  Sum3/1 -> Gain1/1
  in/1 -> Sum3/1
  Gain1/1 -> Saturation1/1
  Saturation1/1 -> Integrator/1

== system My_gfm_battery_sil_2_2/My Inverter Controller 1/My_machineModel_A/governer/synchronizer/HPF  ==
  in : Inport
  Integrator : Integrator
  Sum : Sum  Inputs=|+-
  wSync : Gain  Gain=wSync
  out : Outport  VectorParamsAs1DForOutWhenUnconnected=on
  wires:
  Sum/1 -> out/1, wSync/1
  in/1 -> Sum/1
  Integrator/1 -> Sum/2
  wSync/1 -> Integrator/1

== system My_gfm_battery_sil_2_2/My Inverter Controller 1/My_machineModel_A/governer/synchronizer/assymmetric filter1 ==
  note: The saturation block is configured to cause a rapid rise, but much slow drop in output.
  in : Inport
  Gain1 : Gain  Gain=1/tauBkSt
  Integrator : Integrator
  Saturation1 : Saturate  UpperLimit=VllRated  LowerLimit=-0.02 * VllRated
  Sum3 : Sum  Inputs=|+-
  out : Outport  VectorParamsAs1DForOutWhenUnconnected=on
  wires:
  Integrator/1 -> out/1, Sum3/2
  Sum3/1 -> Gain1/1
  in/1 -> Sum3/1
  Gain1/1 -> Saturation1/1
  Saturation1/1 -> Integrator/1

== system My_gfm_battery_sil_2_2/My Inverter Controller 1/My_machineModel_A1/governer/synchronizer/HPF ==
  in : Inport
  1/tau : Gain  Gain=2*pi*50
  Integrator : Integrator
  Sum : Sum  Inputs=|+-
  out : Outport  VectorParamsAs1DForOutWhenUnconnected=on
  wires:
  Sum/1 -> out/1, 1/tau/1
  in/1 -> Sum/1
  Integrator/1 -> Sum/2
  1/tau/1 -> Integrator/1

== system My_gfm_battery_sil_2_2/My Inverter Controller 1/My_machineModel_A1/governer/synchronizer/assymmetric filter1 ==
  note: The saturation block is configured to cause a rapid rise, but much slow drop in output.
  in : Inport
  Gain1 : Gain  Gain=2
  Integrator : Integrator
  Saturation1 : Saturate  UpperLimit=VllRated  LowerLimit=-0.02 * VllRated
  Sum3 : Sum  Inputs=|+-
  out : Outport  VectorParamsAs1DForOutWhenUnconnected=on
  wires:
  Integrator/1 -> out/1, Sum3/2
  Sum3/1 -> Gain1/1
  in/1 -> Sum3/1
  Gain1/1 -> Saturation1/1
  Saturation1/1 -> Integrator/1

== system My_gfm_battery_sil_2_2/My Inverter Controller 1/My_machineModel_A1/governer1/synchronizer/HPF ==
  in : Inport
  1/tau : Gain  Gain=2*pi*50
  Integrator : Integrator
  Sum : Sum  Inputs=|+-
  out : Outport  VectorParamsAs1DForOutWhenUnconnected=on
  wires:
  Sum/1 -> out/1, 1/tau/1
  in/1 -> Sum/1
  Integrator/1 -> Sum/2
  1/tau/1 -> Integrator/1

== system My_gfm_battery_sil_2_2/My Inverter Controller 1/My_machineModel_A1/governer1/synchronizer/assymmetric filter1 ==
  note: The saturation block is configured to cause a rapid rise, but much slow drop in output.
  in : Inport
  Gain1 : Gain  Gain=2
  Integrator : Integrator
  Saturation1 : Saturate  UpperLimit=VllRated  LowerLimit=-0.02 * VllRated
  Sum3 : Sum  Inputs=|+-
  out : Outport  VectorParamsAs1DForOutWhenUnconnected=on
  wires:
  Integrator/1 -> out/1, Sum3/2
  Sum3/1 -> Gain1/1
  in/1 -> Sum3/1
  Gain1/1 -> Saturation1/1
  Saturation1/1 -> Integrator/1
